simulink model "FSEA_Vehicle"  (R2026a)
settings: Solver=ode23tb  StopTime=5  FixedStep=.001  RelTol=1e-1
model workspace (MAT data in the model file):
  A_mu = 10
  B_reff = 8.386
  CONVERTER_DATA = [0 0.1 0.2 0.3 0.4 0.5 0.6 0.7 0.8 0.81 0.82 0.83 ... (63 elements, 21x3)]
  Cps = 2
  Cz = 7766.25
  DOWN_TABLE = [0 0 0 0 0 0 5 5 7.5 7.5 15 15 ... (30 elements, 6x5)]
  DOWN_TH_BP = [0 5 40 50 90 100]
  D_reff = 0.25826
  EMAP = [-40 215 245 264 264 267 267 267 267 267 -44 117 ... (110 elements, 10x11)]
  F0z = [6086.4 4324.8]
  F_reff = 0.07394
  F_zmax = 10000
  F_zmin = 100
  F_zo = 4000
  Kz = 48000
  MF : object (value not decoded)
  NCyl = 6
  NE_VEC = [800 1200 1600 2000 2400 2800 3200 3600 4000 4400 4800]
  Pstd = 101325
  Rair = 287
  SUS : object (value not decoded)
  TH_VEC = [0; 20; 30; 40; 50; 60; 70; 80; 90; 100]
  TWAITdn = 1.25
  TWAITup = 0.1
  Tin = [1 2 3 4 5 6 7 8 9 10 2 2 ... (20 elements, 10x2)]
  Tstd = 293.15
  UP_TABLE = [7.5 7.5 15 25 40 40 25 25 35 45 70 80 ... (30 elements, 6x5)]
  UP_TH_BP = [0 25 35 50 90 100]
  VEH : object (value not decoded)
  V_o = 16.7
  V_xlow = 1
  Vd = 0.00346
  WH : object (value not decoded)
  a = 1.515
  alpha_max = 1.5
  alpha_min = -1.5
  b = 1.504
  c_zo = 209651
  epsilon = 0.1
  f_air = [0 0 0 0 0 0 0 0 0 0 0 0 ... (256 elements, 16x16)]
  f_co = [0 0 0 0 0 0 0 0 0 0 0 0 ... (256 elements, 16x16)]
  f_co2 = [0 0 0 0 0 0 0 0 0 0 0 0 ... (256 elements, 16x16)]
  f_eff = [352.135682859 352.135682859 320.724378192 303.655312657 295.930136708 291.240087194 291.240271258 291.240312459 291.240275452 291.240198499 291.240100781 291.240018769 ... (256 elements, 16x16)]
  f_fuel = [0 0 0 0 0 0 0 0 0 0 0 0 ... (256 elements, 16x16)]
  f_hc = [0 0 0 0 0 0 0 0 0 0 0 0 ... (256 elements, 16x16)]
  f_nox = [0 0 0 0 0 0 0 0 0 0 0 0 ... (256 elements, 16x16)]
  f_pm = [0 0 0 0 0 0 0 0 0 0 0 0 ... (256 elements, 16x16)]
  f_susp_axl_bp = [1 2]
  f_susp_dz_bp = [-4 -0.14 -0.13 -0.12 -0.11 -0.1 -0.09 -0.08 -0.07 -0.06 -0.05 -0.04 ... (31 elements, 1x31)]
  f_susp_dzdot_bp = [-4 -0.14 -0.13 -0.12 -0.11 -0.1 -0.09 -0.08 -0.07 -0.06 -0.05 -0.04 ... (31 elements, 1x31)]
  f_susp_fmz = [-213379.591456 -28099.591456 -27619.591456 -27139.591456 -26659.591456 -26179.591456 -25699.591456 -25219.591456 -24739.591456 -24259.591456 -23779.591456 -23299.591456 ... (468968 elements, 31x31x61x2x4)]
  f_susp_geom = [-0.832564012244 0.043269987756 0.045538987756 0.047807987756 0.050076987756 0.052345987756 0.054614987756 0.056883987756 0.059152987756 0.061421987756 0.063690987756 0.065959987756 ... (11346 elements, 31x61x2x3)]
  f_susp_strgdelta_bp = [-0.523598775598 -0.506145483078 -0.488692190558 -0.471238898038 -0.453785605519 -0.436332312999 -0.418879020479 -0.401425727959 -0.383972435439 -0.366519142919 -0.349065850399 -0.331612557879 ... (61 elements, 1x61)]
  f_tbrake = [0 76.8593923996 105.140482948 131.533638111 157.926793274 176.658631717 176.65727296 176.656856686 176.656879077 176.657093756 176.657404516 176.65772406 ... (256 elements, 16x16)]
  f_tbrake_n_bpt = [0 649.519052838 912.419621844 1175.32019085 1438.22075986 1701.12132886 1964.02189787 2226.92246687 2489.82303588 2752.72360489 3015.62417389 3278.5247429 ... (16 elements, 1x16)]
  f_tbrake_t_bpt = [0 34.6410161514 61.0341713143 87.4273264773 113.82048164 140.213636803 166.606791966 192.999947129 219.393102292 245.786257455 272.179412618 298.572567781 ... (16 elements, 1x16)]
  f_texh = [766.752464599 766.752464599 786.17542386 801.679939032 884.591982581 910.574397722 910.571871054 910.570774534 910.570601632 910.570821151 910.571247242 910.571639815 ... (256 elements, 16x16)]
  f_twc_eff_co = [0.17 0.25 0.45 0.99 0.99 0.99 0.99]
  f_twc_eff_hc = [0.21 0.375 0.75 0.98 0.98 0.98 0.98]
  f_twc_eff_lam = [0.909090909 0.944055944 0.979020979 1 1.013986014 1.048951049 1.083916084]
  f_twc_eff_nox = [0.98 0.98 0.98 0.97 0.05 0.02 0]
  h = 0.134
  k_z = 50
  kappa_max = 1.5
  kappa_min = -1.5
  lam_Cx = 1
  lam_Cy = 1
  lam_Cz = 1
  lam_Ex = 1
  lam_Ey = 1
  lam_F_zo = 1
  lam_Hx = 1
  lam_Hy = 1
  lam_Kxkappa = 1
  lam_Kyalpha = 1
  lam_Kygamma = 1
  lam_Kzgamma = 1
  lam_Mr = 1
  lam_Mx = 1
  lam_My = 1
  lam_S = 1
  lam_VMx = 1
  lam_Vx = 1
  lam_Vy = 1
  lam_Vykappa = 1
  lam_muV = 0
  lam_mux = 1
  lam_muy = 1
  lam_t = 1
  lam_xalpha = 1
  lam_ykappa = 1
  numWheel = 4
  p_Cx1 = 1.579
  p_Cy1 = 1.3332
  p_Dx1 = 1.0422
  p_Dx2 = -0.08285
  p_Dx3 = 0
  p_Dy1 = 0.8784
  p_Dy2 = -0.06445
  p_Dy3 = 0
  p_Ex1 = 0.11185
  p_Ex2 = 0.3127
  p_Ex3 = 0
  p_Ex4 = 0.001603
  p_Ey1 = -0.8227
  p_Ey2 = -0.6062
  p_Ey3 = 0.09825
  p_Ey4 = -6.546
  p_Ey5 = 0
  p_Fz1 = 0.7098
  p_Hx1 = 0.00021585
  p_Hx2 = 0.0011538
  p_Hy1 = -0.0018043
  p_Hy2 = 0.003518
  p_Kx1 = 21.69
  p_Kx2 = 13.774
  p_Kx3 = -0.4119
  p_Ky1 = -15.314
  p_Ky2 = 1.7044
  p_Ky3 = 0.36986
  p_Ky4 = 1.9896
  p_Ky5 = 0
  p_Ky6 = -0.9004
  p_Ky7 = -0.2328
  p_Vx1 = 1.5973e-05
  p_Vx2 = 0.0001043
  p_Vy1 = -0.006642
  p_Vy2 = 0.03597
  p_Vy3 = -0.1621
  p_Vy4 = -0.4908
  p_pmx1 = 0
  p_px1 = -0.3489
  p_px2 = 0.382
  p_px3 = -0.09634
  p_px4 = 0.06447
  p_py1 = -0.6249
  p_py2 = -0.06535
  p_py3 = -0.1668
  p_py4 = 0.2834
  p_py5 = 0
  path : object (value not decoded)
  pio = 220000
  q_Fcx = 0
  q_Fz2 = 15.4
  q_Fzy = 0
  q_reo = 0.9974
  q_sx1 = -0.007764
  q_sx10 = 0.2824
  q_sx11 = 5.349
  q_sx12 = 0
  q_sx13 = 0
  q_sx14 = 0
  q_sx2 = 1.1915
  q_sx3 = 0.013948
  q_sx4 = 4.912
  q_sx5 = 1.02
  q_sx6 = 22.83
  q_sx7 = 0.7104
  q_sx8 = -0.023393
  q_sx9 = 0.6581
  q_sy1 = 0.00702
  q_sy2 = 0
  q_sy3 = 0.001515
  q_sy4 = 8.514e-05
  q_sy5 = 0
  q_sy6 = 0
  q_sy7 = 0.9008
  q_sy8 = -0.4089
  q_v1 = 0.0007742
  q_v2 = 0.04667
  r_Bx1 = 12.531
  r_Bx2 = 9.532
  r_Bx3 = 0
  r_By1 = 10.615
  r_By2 = 7.705
  r_By3 = 3.433e-06
  r_By4 = 0
  r_Cx1 = 1.019
  r_Cy1 = 1.0585
  r_Ex1 = -0.4487
  r_Ex2 = -0.4726
  r_Ey1 = 0.3132
  r_Ey2 = 7.63e-06
  r_Hx1 = 0.0002374
  r_Hy1 = 0.011646
  r_Hy2 = 7.63e-06
  r_Vy1 = 0.05654
  r_Vy2 = 7.63e-06
  r_Vy3 = 0
  r_Vy4 = 99.9
  r_Vy5 = 2
  r_Vy6 = 15.814
  r_o = 0.3135
  reqTmaxT = [nan 0.285774810084 0.647179872268 nan nan nan nan nan nan nan nan nan ... (168 elements, 21x8)]
  vehSpd = [0 2.77777777778 5.55555555556 8.33333333333 11.1111111111 13.8888888889 16.6666666667 19.4444444444 22.2222222222 25 27.7777777778 30.5555555556 ... (21 elements, 1x21)]
  vehWidth = 2
  w = 1
symbols that are objects in the model workspace (value not decoded): VEH
undefined symbols (not defined in the file or in its folder): InertFrm
libraries: sharedtransform x6, vehdynlibtirecommon x2, vehdynlibtire x2, autolibutils x2, autolibshared x2
(part 3 of 4)

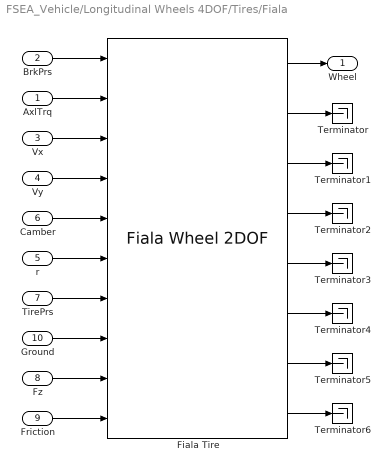
== system FSEA_Vehicle/Longitudinal Wheels 4DOF/Tires/Fiala ==
  AxlTrq : Inport
  BrkPrs : Inport  Port=2
  Vx : Inport  Port=3
  Vy : Inport  Port=4
  r : Inport  Port=5
  Camber : Inport  Port=6
  TirePrs : Inport  Port=7
  Fz : Inport  Port=8
  Friction : Inport  Port=9
  Ground : Inport  Port=10
  Fiala Tire : vehdynlibtire/Fiala Wheel 2DOF  tireType=Mid-size passenger car 235/45R18  BrakeType=Disc  rollingType=Pressure and velocity  vertType=None  Ckappa=217325.388  Calpha=104298.5693  Cgamma=-3413.1559  muMin=0.17601  muMax=1.3803  Lrelx=.01  Lrely=.01  NOMPRES=220000  LONGVL=16  aMy=8e-4  bMy=.001  cMy=1.6e-4  alphaMy=-0.003  betaMy=0.97  QSY1=0.007  QSY2=0  QSY3=0.0015  QSY4=8.5e-05  QSY5=0  QSY6=0  QSY7=0.9  QSY8=-0.4  FNOMIN=4000  lam_My=1  VxMy=-20:1:20  FzMy=0:200:1e4  MyMap=|  Fpl=10  Cr=1e-3  Kt=.008  Tmeas=298.15  Tamb=298.15  extTamb=off  WIDTH=0.235  bMz=0  mu_static=.3  mu_kinetic=.2  disk_abore=.05  Rm=.177  num_pads=2  drum_abore=0.0508  drum_a=0.123  drum_c=0.212  drum_r=0.15  drum_theta1=0  drum_theta2=126  brake_p_bpt=[1 11.4736842105263 21.9473684210526 32.4210526315789 42.8947368421053 53.3684210526316 63.8421052631579 74.3157894736842 84.7894736842105 95.2631578947368 105.736842105263 116.210526315789 126.684210526316 137.157894736842 147.631578947368 158.105263157895 168.578947368421 179.052631578947 189.526315789474 200]  brake_n_bpt=[0 52.6315789473684 105.263157894737 157.894736842105 210.526315789474 263.157894736842 315.789473684211 368.421052631579 421.052631578947 473.684210526316 526.315789473684 578.947368421053 631.578947368421 684.210526315789 736.842105263158 789.473684210526 842.105263157895 894.736842105263 947.368421052632 1000]  f_brake_t=[43.4900602404453 42.5056030554862 41.5350898940194 40.5780454442085 39.6340111501808 38.7025443887544 37.7832176914519 36.8756180088306 35.9793460143796 35.0940154454303 34.2192524787115 33.3546951383474 32.4999927342521 31.6548053290159 30.8188032315107 29.991666515561 29.1730845621415 28.362755623661 27.5603864089927 26.765691687993;498.991217495636 487.695866636631 476.560505099801 465.579679307235 454.748127933653 444.060772460445 433.51270824929 423.099196101319 412.81565427025 402.657650900201 392.620896861006 382.701238955775 372.894653477208 363.197240090814 353.605216024701 344.114910546964 334.722759712992 325.425301366216 316.219170376863 307.10109410434;954.492374750826 932.886130217776 911.585920305583 890.581313170261 869.862244717126 849.419000532136 829.242198807128 809.322774193808 789.651962526121 770.221286354971 751.0225412433 732.047782773203 713.289314220164 694.739674852612 676.391628817892 658.238154578366 640.272434863842 622.48784710877 604.877954344734 587.436496520688;1409.99353200602 1378.07639379892 1346.61133551136 1315.58294703329 1284.9763615006 1254.77722860383 1224.97168936497 1195.5463522863 1166.48827078199 1137.78492180974 1109.42418562559 1081.39432659063 1053.68397496312 1026.28210961441 999.178041611083 972.361398609768 945.822110014692 919.550392851325 893.536738312604 867.771898937035;1865.49468926121 1823.26665738007 1781.63675071715 1740.58458089631 1700.09047828407 1660.13545667552 1620.7011799228 1581.76993037878 1543.32457903786 1505.34855726451 1467.82583000789 1430.74087040806 1394.07863570608 1357.82454437621 1321.96445440427 1286.48464264117 1251.37178516554 1216.61293859388 1182.19552228048 1148.10730135338;2320.9958465164 2268.45692096121 2216.66216592293 2165.58621475934 2115.20459506754 2065.49368474721 2016.43067048064 1967.99350847127 1920.16088729373 1872.91219271928 1826.22747439018 1780.08741422549 1734.47329644903 1689.36697913801 1644.75086719747 1600.60788667257 1556.92146031639 1513.67548433643 1470.85430624835 1428.44270376973;2776.49700377159 2713.64718454235 2651.68758112871 2590.58784862237 2530.31871185102 2470.8519128189 2412.16016103848 2354.21708656376 2296.9971955496 2240.47582817405 2184.62911877248 2129.43395804292 2074.86795719199 2020.9094138998 1967.53727999066 1914.73113070398 1862.47113546724 1810.73803007899 1759.51309021622 1708.77810618608;3231.99816102678 3158.8374481235 3086.71299633449 3015.58948248539 2945.43282863449 2876.21014089059 2807.88965159632 2740.44066465625 2673.83350380547 2608.03946362882 2543.03076315477 2478.78050186034 2415.26261793494 2352.4518486616 2290.32369278385 2228.85437473538 2168.02081061809 2107.80057582154 2048.17187418409 1989.11350860242;3687.49931828197 3604.02771170464 3521.73841154027 3440.59111634842 3360.54694541796 3281.56836896228 3203.61914215416 3126.66424274874 3050.66981206134 2975.60309908359 2901.43240753707 2828.12704567777 2755.6572786779 2683.9942834234 2613.11010557704 2542.97761876678 2473.57048576894 2404.8631215641 2336.83065815196 2269.44891101877;4143.00047553716 4049.21797528579 3956.76382674606 3865.59275021144 3775.66106220143 3686.92659703397 3599.34863271199 3512.88782084123 3427.50612031721 3343.16673453836 3259.83405191936 3177.4735894952 3096.05193942085 3015.5367181852 2935.89651837023 2857.10086279818 2779.12016091979 2701.92566730665 2625.48944211983 2549.78431343512;4598.50163279235 4494.40823886693 4391.78924195184 4290.59438407447 4190.77517898491 4092.28482510566 3995.07812326983 3899.11139893372 3804.34242857308 3710.73036999313 3618.23569630166 3526.82013331263 3436.44660016381 3347.079152947 3258.68293116342 3171.22410682959 3084.66983607064 2998.98821304921 2914.1482260877 2830.11971585147;5054.00279004754 4939.59850244808 4826.81465715762 4715.59601793749 4605.88929576838 4497.64305317735 4390.80761382767 4285.3349770262 4181.17873682896 4078.2940054479 3976.63734068395 3876.16667713006 3776.84126090677 3678.62158770879 3581.46934395661 3485.34735086099 ...(+2764 chars)]  MASS=9.46491996974568  zo=0  zdoto=0  GRAVITY=-9.81  VERTICAL_STIFFNESS=207885  VERTICAL_DAMPING=500  zFz=[0 .01 .1]  pFz=[10000 1000000]  Fzz=[0 1e3 1e4; 0 1e4 1e5]  zdotFz=[-20 0 20]  Fzzdot=[500 0 -500;250 0 -250]  UNLOADED_RADIUS=0.33454  omegao=0  IYY=0.740633832792491  br=1e-3  FZMAX=8600  FZMIN=100  PRESMAX=1000000  PRESMIN=10000  KPUMAX=0.5  KPUMIN=-0.5  ALPMAX=0.7854  ALPMIN=-0.7854  CAMMAX=0.17453  CAMMIN=-0.17453  TMIN=0  TMAX=400  aMode=2  MyRelFreqLwrLim=100*pi
      | [0,1114.7,4367.1,9707.2,17109,26554,38030,51524,67028,84533,1.0403e+05,1.2552e+05,1.4899e+05,1.7444e+05,2.0185e+05,2.3124e+05,2.6259e+05,2.959e+05,3.3117e+05,3.6839e+05,4.0756e+05,4.4868e+05,4.9174e+05,5.3675e+05,5.8369e+05,6.3257e+05,6.8338e+05,7.3613e+05,7.908e+05,8.474e+05,9.0593e+05,9.6638e+05,1.0288e+06,1.093e+06,1.1593e+06,1.2274e+06,1.2974e+06,1.3694e+06,1.4432e+06,1.519e+06,1.5967e+06,1.6763e+06,1.7578e+06,1.8412e+06,1.9265e+06,2.0137e+06,2.1028e+06,2.1938e+06,2.2867e+06,2.3815e+06,2.4782e+06
      | 0,1024.5,4013.8,8921.9,15725,24406,34953,47356,61605,77694,95616,1.1537e+05,1.3694e+05,1.6032e+05,1.8553e+05,2.1254e+05,2.4135e+05,2.7197e+05,3.0438e+05,3.3859e+05,3.7459e+05,4.1238e+05,4.5196e+05,4.9333e+05,5.3647e+05,5.814e+05,6.281e+05,6.7658e+05,7.2683e+05,7.7885e+05,8.3264e+05,8.8821e+05,9.4553e+05,1.0046e+06,1.0655e+06,1.1281e+06,1.1925e+06,1.2586e+06,1.3265e+06,1.3961e+06,1.4675e+06,1.5407e+06,1.6156e+06,1.6922e+06,1.7706e+06,1.8508e+06,1.9327e+06,2.0163e+06,2.1017e+06,2.1889e+06,2.2777e+06
      | 0,938.57,3677,8173.3,14405,22358,32020,43382,56436,71175,87593,1.0568e+05,1.2545e+05,1.4687e+05,1.6996e+05,1.947e+05,2.211e+05,2.4915e+05,2.7884e+05,3.1018e+05,3.4316e+05,3.7778e+05,4.1404e+05,4.5193e+05,4.9146e+05,5.3261e+05,5.754e+05,6.1981e+05,6.6584e+05,7.135e+05,7.6278e+05,8.1368e+05,8.6619e+05,9.2032e+05,9.7607e+05,1.0334e+06,1.0924e+06,1.153e+06,1.2152e+06,1.279e+06,1.3444e+06,1.4114e+06,1.48e+06,1.5502e+06,1.6221e+06,1.6955e+06,1.7705e+06,1.8471e+06,1.9254e+06,2.0052e+06,2.0866e+06
      | 0,856.81,3356.7,7461.3,13151,20411,29231,39603,51520,64974,79962,96478,1.1452e+05,1.3408e+05,1.5515e+05,1.7774e+05,2.0184e+05,2.2744e+05,2.5455e+05,2.8316e+05,3.1327e+05,3.4487e+05,3.7797e+05,4.1256e+05,4.4864e+05,4.8621e+05,5.2527e+05,5.6581e+05,6.0784e+05,6.5134e+05,6.9633e+05,7.4279e+05,7.9073e+05,8.4015e+05,8.9104e+05,9.4341e+05,9.9724e+05,1.0525e+06,1.1093e+06,1.1676e+06,1.2273e+06,1.2885e+06,1.3511e+06,1.4152e+06,1.4808e+06,1.5478e+06,1.6163e+06,1.6862e+06,1.7576e+06,1.8305e+06,1.9048e+06
      | 0,779.25,3052.9,6785.9,11960,18563,26585,36018,46856,59093,72724,87745,1.0415e+05,1.2194e+05,1.4111e+05,1.6165e+05,1.8357e+05,2.0685e+05,2.3151e+05,2.5753e+05,2.8491e+05,3.1365e+05,3.4376e+05,3.7522e+05,4.0803e+05,4.422e+05,4.7772e+05,5.1459e+05,5.5282e+05,5.9238e+05,6.333e+05,6.7556e+05,7.1916e+05,7.641e+05,8.1039e+05,8.5801e+05,9.0697e+05,9.5727e+05,1.0089e+06,1.0619e+06,1.1162e+06,1.1718e+06,1.2288e+06,1.2871e+06,1.3467e+06,1.4077e+06,1.47e+06,1.5336e+06,1.5985e+06,1.6648e+06,1.7324e+06
      | 0,705.9,2765.5,6147.1,10834,16816,24083,32628,42446,53531,65879,79486,94348,1.1046e+05,1.2783e+05,1.4643e+05,1.6629e+05,1.8738e+05,2.0972e+05,2.3329e+05,2.5809e+05,2.8413e+05,3.114e+05,3.399e+05,3.6962e+05,4.0058e+05,4.3276e+05,4.6616e+05,5.0078e+05,5.3662e+05,5.7369e+05,6.1197e+05,6.5146e+05,6.9218e+05,7.3411e+05,7.7725e+05,8.216e+05,8.6717e+05,9.1394e+05,9.6193e+05,1.0111e+06,1.0615e+06,1.1131e+06,1.1659e+06,1.22e+06,1.2752e+06,1.3316e+06,1.3892e+06,1.4481e+06,1.5081e+06,1.5693e+06
      | 0,636.76,2494.6,5545,9773.1,15169,21724,29432,38288,48287,59426,71700,85106,99642,1.153e+05,1.3209e+05,1.5e+05,1.6903e+05,1.8917e+05,2.1044e+05,2.3281e+05,2.563e+05,2.809e+05,3.066e+05,3.3342e+05,3.6134e+05,3.9037e+05,4.205e+05,4.5173e+05,4.8406e+05,5.1749e+05,5.5202e+05,5.8765e+05,6.2438e+05,6.622e+05,7.0111e+05,7.4112e+05,7.8223e+05,8.2442e+05,8.677e+05,9.1208e+05,9.5754e+05,1.0041e+06,1.0517e+06,1.1005e+06,1.1503e+06,1.2012e+06,1.2532e+06,1.3062e+06,1.3604e+06,1.4156e+06
      | 0,571.82,2240.2,4979.5,8776.4,13622,19508,26430,34383,43363,53365,64388,76427,89480,1.0355e+05,1.1862e+05,1.347e+05,1.5179e+05,1.6988e+05,1.8897e+05,2.0907e+05,2.3016e+05,2.5225e+05,2.7534e+05,2.9942e+05,3.2449e+05,3.5056e+05,3.7761e+05,4.0566e+05,4.3469e+05,4.6472e+05,4.9573e+05,5.2772e+05,5.607e+05,5.9467e+05,6.2961e+05,6.6554e+05,7.0245e+05,7.4034e+05,7.7921e+05,8.1906e+05,8.5989e+05,9.017e+05,9.4448e+05,9.8824e+05,1.033e+06,1.0787e+06,1.1254e+06,1.173e+06,1.2216e+06,1.2712e+06
      | 0,511.09,2002.3,4450.7,7844.3,12175,17436,23623,30732,38757,47698,57549,68310,79977,92548,1.0602e+05,1.204e+05,1.3567e+05,1.5184e+05,1.689e+05,1.8686e+05,2.0572e+05,2.2546e+05,2.4609e+05,2.6762e+05,2.9003e+05,3.1332e+05,3.3751e+05,3.6258e+05,3.8853e+05,4.1536e+05,4.4308e+05,4.7167e+05,5.0115e+05,5.3151e+05,5.6274e+05,5.9486e+05,6.2785e+05,6.6171e+05,6.9646e+05,7.3207e+05,7.6857e+05,8.0593e+05,8.4417e+05,8.8328e+05,9.2326e+05,9.6412e+05,1.0058e+06,1.0484e+06,1.0919e+06,1.1362e+06
      | 0,454.56,1780.8,3958.4,6976.8,10828,15508,21011,27333,34471,42422,51185,60755,71132,82313,94296,1.0708e+05,1.2066e+05,1.3505e+05,1.5022e+05,1.662e+05,1.8296e+05,2.0052e+05,2.1888e+05,2.3802e+05,2.5795e+05,2.7867e+05,3.0018e+05,3.2248e+05,3.4556e+05,3.6942e+05,3.9407e+05,4.1951e+05,4.4573e+05,4.7273e+05,5.0051e+05,5.2907e+05,5.5841e+05,5.8853e+05,6.1943e+05,6.5111e+05,6.8356e+05,7.168e+05,7.5081e+05,7.8559e+05,8.2115e+05,8.5749e+05,8.946e+05,9.3248e+05,9.7114e+05,1.0106e+06
      | 0,402.25,1575.9,3502.8,6173.8,9582.1,13723,18592,24187,30503,37540,45293,53762,62945,72839,83443,94756,1.0678e+05,1.195e+05,1.3293e+05,1.4707e+05,1.6191e+05,1.7745e+05,1.9368e+05,2.1062e+05,2.2826e+05,2.466e+05,2.6563e+05,2.8536e+05,3.0578e+05,3.269e+05,3.4872e+05,3.7123e+05,3.9442e+05,4.1832e+05,4.429e+05,4.6817e+05,4.9414e+05,5.2079e+05,5.4814e+05,5.7617e+05,6.0489e+05,6.343e+05,6.6439e+05,6.9517e+05,7.2664e+05,7.588e+05,7.9163e+05,8.2516e+05,8.5937e+05,8.9426e+05
      | 0,354.13,1387.4,3083.9,5435.3,8436,12082,16369,21294,26855,33050,39876,47332,55416,64127,73463,83423,94005,1.0521e+05,1.1703e+05,1.2948e+05,1.4254e+05,1.5622e+05,1.7052e+05,1.8543e+05,2.0096e+05,2.171e+05,2.3386e+05,2.5123e+05,2.6921e+05,2.878e+05,3.0701e+05,3.2682e+05,3.4725e+05,3.6828e+05,3.8993e+05,4.1218e+05,4.3504e+05,4.585e+05,4.8258e+05,5.0725e+05,5.3254e+05,5.5843e+05,5.8493e+05,6.1203e+05,6.3973e+05,6.6804e+05,6.9695e+05,7.2646e+05,7.5658e+05,7.873e+05
      | 0,310.23,1215.4,2701.5,4761.5,7390.2,10584,14339,18654,23526,28952,34932,41464,48546,56176,64355,73080,82351,92166,1.0252e+05,1.1343e+05,1.2487e+05,1.3685e+05,1.4938e+05,1.6244e+05,1.7605e+05,1.9019e+05,2.0487e+05,2.2008e+05,2.3583e+05,2.5212e+05,2.6895e+05,2.863e+05,3.042e+05,3.2262e+05,3.4158e+05,3.6108e+05,3.811e+05,4.0166e+05,4.2275e+05,4.4437e+05,4.6652e+05,4.892e+05,5.1241e+05,5.3615e+05,5.6042e+05,5.8521e+05,6.1054e+05,6.364e+05,6.6278e+05,6.8969e+05
      | 0,270.53,1059.9,2355.8,4152.2,6444.5,9229.4,12504,16267,20515,25247,30462,36158,42334,48988,56120,63728,71813,80372,89405,98911,1.0889e+05,1.1934e+05,1.3026e+05,1.4166e+05,1.5352e+05,1.6585e+05,1.7865e+05,1.9192e+05,2.0566e+05,2.1986e+05,2.3453e+05,2.4967e+05,2.6527e+05,2.8134e+05,2.9787e+05,3.1487e+05,3.3233e+05,3.5026e+05,3.6865e+05,3.875e+05,4.0682e+05,4.266e+05,4.4684e+05,4.6754e+05,4.887e+05,5.1033e+05,5.3241e+05,5.5496e+05,5.7797e+05,6.0143e+05
      | 0,235.04,920.8,2046.8,3607.4,5599,8018.6,10864,14133,17824,21935,26466,31414,36780,42561,48757,55367,62391,69827,77675,85934,94604,1.0368e+05,1.1317e+05,1.2307e+05,1.3338e+05,1.4409e+05,1.5521e+05,1.6674e+05,1.7867e+05,1.9101e+05,2.0376e+05,2.1691e+05,2.3047e+05,2.4443e+05,2.5879e+05,2.7356e+05,2.8873e+05,3.0431e+05,3.2028e+05,3.3666e+05,3.5345e+05,3.7063e+05,3.8821e+05,4.062e+05,4.2459e+05,4.4337e+05,4.6256e+05,4.8215e+05,5.0214e+05,5.2253e+05
      | 0,203.75,798.24,1774.3,3127.2,4853.7,6951.2,9417.7,12252,15451,19015,22943,27233,31884,36896,42267,47997,54086,60533,67336,74496,82011,89882,98108,1.0669e+05,1.1562e+05,1.2491e+05,1.3455e+05,1.4455e+05,1.5489e+05,1.6559e+05,1.7664e+05,1.8804e+05,1.9979e+05,2.1189e+05,2.2434e+05,2.3715e+05,2.503e+05,2.638e+05,2.7765e+05,2.9185e+05,3.064e+05,3.2129e+05,3.3654e+05,3.5213e+05,3.6807e+05,3.8436e+05,4.0099e+05,4.1797e+05,4.353e+05,4.5297e+05
      | 0,176.67,692.15,1538.5,2711.6,4208.6,6027.4,8166.1,10623,13398,16488,19894,23613,27646,31992,36650,41618,46898,52488,58387,64595,71112,77937,85069,92509,1.0026e+05,1.0831e+05,1.1667e+05,1.2533e+05,1.3431e+05,1.4358e+05,1.5316e+05,1.6305e+05,1.7324e+05,1.8373e+05,1.9453e+05,2.0563e+05,2.1703e+05,2.2874e+05,2.4075e+05,2.5306e+05,2.6568e+05,2.7859e+05,2.9181e+05,3.0533e+05,3.1915e+05,3.3327e+05,3.477e+05,3.6242e+05,3.7745e+05,3.9277e+05
      | 0,153.8,602.54,1339.3,2360.6,3663.8,5247,7108.9,9247.9,11663,14353,17318,20556,24067,27850,31905,36230,40826,45692,50828,56232,61905,67847,74056,80533,87277,94287,1.0156e+05,1.0911e+05,1.1692e+05,1.2499e+05,1.3333e+05,1.4194e+05,1.5081e+05,1.5994e+05,1.6934e+05,1.7901e+05,1.8894e+05,1.9913e+05,2.0958e+05,2.203e+05,2.3128e+05,2.4253e+05,2.5403e+05,2.658e+05,2.7783e+05,2.9013e+05,3.0268e+05,3.155e+05,3.2858e+05,3.4192e+05
      | 0,135.13,529.41,1176.8,2074.1,3219.1,4610.2,6246.1,8125.5,10248,12611,15216,18061,21146,24470,28033,31833,35871,40147,44659,49407,54392,59612,65068,70759,76684,82844,89238,95866,1.0273e+05,1.0982e+05,1.1715e+05,1.2471e+05,1.3251e+05,1.4053e+05,1.4879e+05,1.5728e+05,1.66e+05,1.7496e+05,1.8415e+05,1.9356e+05,2.0321e+05,2.1309e+05,2.232e+05,2.3354e+05,2.4411e+05,2.5492e+05,2.6595e+05,2.7721e+05,2.887e+05,3.0042e+05
      | 0,120.67,472.76,1050.9,1852.1,2874.6,4116.9,5577.7,7256.1,9151,11262,13588,16129,18883,21852,25033,28427,32033,35851,39880,44121,48572,53234,58105,63187,68479,73979,79689,85608,91735,98071,1.0462e+05,1.1137e+05,1.1833e+05,1.255e+05,1.3287e+05,1.4045e+05,1.4824e+05,1.5624e+05,1.6444e+05,1.7285e+05,1.8147e+05,1.9029e+05,1.9932e+05,2.0855e+05,2.1799e+05,2.2764e+05,2.3749e+05,2.4755e+05,2.5781e+05,2.6828e+05
      | 0,110.42,432.59,961.56,1694.8,2630.4,3767.1,5103.8,6639.5,8373.5,10305,12433,14758,17279,19995,22906,26012,29311,32805,36492,40372,44445,48710,53168,57818,62660,67694,72918,78334,83941,89738,95727,1.019e+05,1.0827e+05,1.1483e+05,1.2158e+05,1.2852e+05,1.3565e+05,1.4296e+05,1.5047e+05,1.5816e+05,1.6605e+05,1.7412e+05,1.8238e+05,1.9083e+05,1.9947e+05,2.083e+05,2.1731e+05,2.2651e+05,2.359e+05,2.4548e+05
      | 0,120.67,472.76,1050.9,1852.1,2874.6,4116.9,5577.7,7256.1,9151,11262,13588,16129,18883,21852,25033,28427,32033,35851,39880,44121,48572,53234,58105,63187,68479,73979,79689,85608,91735,98071,1.0462e+05,1.1137e+05,1.1833e+05,1.255e+05,1.3287e+05,1.4045e+05,1.4824e+05,1.5624e+05,1.6444e+05,1.7285e+05,1.8147e+05,1.9029e+05,1.9932e+05,2.0855e+05,2.1799e+05,2.2764e+05,2.3749e+05,2.4755e+05,2.5781e+05,2.6828e+05
      | 0,135.13,529.41,1176.8,2074.1,3219.1,4610.2,6246.1,8125.5,10248,12611,15216,18061,21146,24470,28033,31833,35871,40147,44659,49407,54392,59612,65068,70759,76684,82844,89238,95866,1.0273e+05,1.0982e+05,1.1715e+05,1.2471e+05,1.3251e+05,1.4053e+05,1.4879e+05,1.5728e+05,1.66e+05,1.7496e+05,1.8415e+05,1.9356e+05,2.0321e+05,2.1309e+05,2.232e+05,2.3354e+05,2.4411e+05,2.5492e+05,2.6595e+05,2.7721e+05,2.887e+05,3.0042e+05
      | 0,153.8,602.54,1339.3,2360.6,3663.8,5247,7108.9,9247.9,11663,14353,17318,20556,24067,27850,31905,36230,40826,45692,50828,56232,61905,67847,74056,80533,87277,94287,1.0156e+05,1.0911e+05,1.1692e+05,1.2499e+05,1.3333e+05,1.4194e+05,1.5081e+05,1.5994e+05,1.6934e+05,1.7901e+05,1.8894e+05,1.9913e+05,2.0958e+05,2.203e+05,2.3128e+05,2.4253e+05,2.5403e+05,2.658e+05,2.7783e+05,2.9013e+05,3.0268e+05,3.155e+05,3.2858e+05,3.4192e+05
      | 0,176.67,692.15,1538.5,2711.6,4208.6,6027.4,8166.1,10623,13398,16488,19894,23613,27646,31992,36650,41618,46898,52488,58387,64595,71112,77937,85069,92509,1.0026e+05,1.0831e+05,1.1667e+05,1.2533e+05,1.3431e+05,1.4358e+05,1.5316e+05,1.6305e+05,1.7324e+05,1.8373e+05,1.9453e+05,2.0563e+05,2.1703e+05,2.2874e+05,2.4075e+05,2.5306e+05,2.6568e+05,2.7859e+05,2.9181e+05,3.0533e+05,3.1915e+05,3.3327e+05,3.477e+05,3.6242e+05,3.7745e+05,3.9277e+05
      | 0,203.75,798.24,1774.3,3127.2,4853.7,6951.2,9417.7,12252,15451,19015,22943,27233,31884,36896,42267,47997,54086,60533,67336,74496,82011,89882,98108,1.0669e+05,1.1562e+05,1.2491e+05,1.3455e+05,1.4455e+05,1.5489e+05,1.6559e+05,1.7664e+05,1.8804e+05,1.9979e+05,2.1189e+05,2.2434e+05,2.3715e+05,2.503e+05,2.638e+05,2.7765e+05,2.9185e+05,3.064e+05,3.2129e+05,3.3654e+05,3.5213e+05,3.6807e+05,3.8436e+05,4.0099e+05,4.1797e+05,4.353e+05,4.5297e+05
      | 0,235.04,920.8,2046.8,3607.4,5599,8018.6,10864,14133,17824,21935,26466,31414,36780,42561,48757,55367,62391,69827,77675,85934,94604,1.0368e+05,1.1317e+05,1.2307e+05,1.3338e+05,1.4409e+05,1.5521e+05,1.6674e+05,1.7867e+05,1.9101e+05,2.0376e+05,2.1691e+05,2.3047e+05,2.4443e+05,2.5879e+05,2.7356e+05,2.8873e+05,3.0431e+05,3.2028e+05,3.3666e+05,3.5345e+05,3.7063e+05,3.8821e+05,4.062e+05,4.2459e+05,4.4337e+05,4.6256e+05,4.8215e+05,5.0214e+05,5.2253e+05
      | 0,270.53,1059.9,2355.8,4152.2,6444.5,9229.4,12504,16267,20515,25247,30462,36158,42334,48988,56120,63728,71813,80372,89405,98911,1.0889e+05,1.1934e+05,1.3026e+05,1.4166e+05,1.5352e+05,1.6585e+05,1.7865e+05,1.9192e+05,2.0566e+05,2.1986e+05,2.3453e+05,2.4967e+05,2.6527e+05,2.8134e+05,2.9787e+05,3.1487e+05,3.3233e+05,3.5026e+05,3.6865e+05,3.875e+05,4.0682e+05,4.266e+05,4.4684e+05,4.6754e+05,4.887e+05,5.1033e+05,5.3241e+05,5.5496e+05,5.7797e+05,6.0143e+05
      | 0,310.23,1215.4,2701.5,4761.5,7390.2,10584,14339,18654,23526,28952,34932,41464,48546,56176,64355,73080,82351,92166,1.0252e+05,1.1343e+05,1.2487e+05,1.3685e+05,1.4938e+05,1.6244e+05,1.7605e+05,1.9019e+05,2.0487e+05,2.2008e+05,2.3583e+05,2.5212e+05,2.6895e+05,2.863e+05,3.042e+05,3.2262e+05,3.4158e+05,3.6108e+05,3.811e+05,4.0166e+05,4.2275e+05,4.4437e+05,4.6652e+05,4.892e+05,5.1241e+05,5.3615e+05,5.6042e+05,5.8521e+05,6.1054e+05,6.364e+05,6.6278e+05,6.8969e+05
      | 0,354.13,1387.4,3083.9,5435.3,8436,12082,16369,21294,26855,33050,39876,47332,55416,64127,73463,83423,94005,1.0521e+05,1.1703e+05,1.2948e+05,1.4254e+05,1.5622e+05,1.7052e+05,1.8543e+05,2.0096e+05,2.171e+05,2.3386e+05,2.5123e+05,2.6921e+05,2.878e+05,3.0701e+05,3.2682e+05,3.4725e+05,3.6828e+05,3.8993e+05,4.1218e+05,4.3504e+05,4.585e+05,4.8258e+05,5.0725e+05,5.3254e+05,5.5843e+05,5.8493e+05,6.1203e+05,6.3973e+05,6.6804e+05,6.9695e+05,7.2646e+05,7.5658e+05,7.873e+05
      | 0,402.25,1575.9,3502.8,6173.8,9582.1,13723,18592,24187,30503,37540,45293,53762,62945,72839,83443,94756,1.0678e+05,1.195e+05,1.3293e+05,1.4707e+05,1.6191e+05,1.7745e+05,1.9368e+05,2.1062e+05,2.2826e+05,2.466e+05,2.6563e+05,2.8536e+05,3.0578e+05,3.269e+05,3.4872e+05,3.7123e+05,3.9442e+05,4.1832e+05,4.429e+05,4.6817e+05,4.9414e+05,5.2079e+05,5.4814e+05,5.7617e+05,6.0489e+05,6.343e+05,6.6439e+05,6.9517e+05,7.2664e+05,7.588e+05,7.9163e+05,8.2516e+05,8.5937e+05,8.9426e+05
      | 0,454.56,1780.8,3958.4,6976.8,10828,15508,21011,27333,34471,42422,51185,60755,71132,82313,94296,1.0708e+05,1.2066e+05,1.3505e+05,1.5022e+05,1.662e+05,1.8296e+05,2.0052e+05,2.1888e+05,2.3802e+05,2.5795e+05,2.7867e+05,3.0018e+05,3.2248e+05,3.4556e+05,3.6942e+05,3.9407e+05,4.1951e+05,4.4573e+05,4.7273e+05,5.0051e+05,5.2907e+05,5.5841e+05,5.8853e+05,6.1943e+05,6.5111e+05,6.8356e+05,7.168e+05,7.5081e+05,7.8559e+05,8.2115e+05,8.5749e+05,8.946e+05,9.3248e+05,9.7114e+05,1.0106e+06
      | 0,511.09,2002.3,4450.7,7844.3,12175,17436,23623,30732,38757,47698,57549,68310,79977,92548,1.0602e+05,1.204e+05,1.3567e+05,1.5184e+05,1.689e+05,1.8686e+05,2.0572e+05,2.2546e+05,2.4609e+05,2.6762e+05,2.9003e+05,3.1332e+05,3.3751e+05,3.6258e+05,3.8853e+05,4.1536e+05,4.4308e+05,4.7167e+05,5.0115e+05,5.3151e+05,5.6274e+05,5.9486e+05,6.2785e+05,6.6171e+05,6.9646e+05,7.3207e+05,7.6857e+05,8.0593e+05,8.4417e+05,8.8328e+05,9.2326e+05,9.6412e+05,1.0058e+06,1.0484e+06,1.0919e+06,1.1362e+06
      | 0,571.82,2240.2,4979.5,8776.4,13622,19508,26430,34383,43363,53365,64388,76427,89480,1.0355e+05,1.1862e+05,1.347e+05,1.5179e+05,1.6988e+05,1.8897e+05,2.0907e+05,2.3016e+05,2.5225e+05,2.7534e+05,2.9942e+05,3.2449e+05,3.5056e+05,3.7761e+05,4.0566e+05,4.3469e+05,4.6472e+05,4.9573e+05,5.2772e+05,5.607e+05,5.9467e+05,6.2961e+05,6.6554e+05,7.0245e+05,7.4034e+05,7.7921e+05,8.1906e+05,8.5989e+05,9.017e+05,9.4448e+05,9.8824e+05,1.033e+06,1.0787e+06,1.1254e+06,1.173e+06,1.2216e+06,1.2712e+06
      | 0,636.76,2494.6,5545,9773.1,15169,21724,29432,38288,48287,59426,71700,85106,99642,1.153e+05,1.3209e+05,1.5e+05,1.6903e+05,1.8917e+05,2.1044e+05,2.3281e+05,2.563e+05,2.809e+05,3.066e+05,3.3342e+05,3.6134e+05,3.9037e+05,4.205e+05,4.5173e+05,4.8406e+05,5.1749e+05,5.5202e+05,5.8765e+05,6.2438e+05,6.622e+05,7.0111e+05,7.4112e+05,7.8223e+05,8.2442e+05,8.677e+05,9.1208e+05,9.5754e+05,1.0041e+06,1.0517e+06,1.1005e+06,1.1503e+06,1.2012e+06,1.2532e+06,1.3062e+06,1.3604e+06,1.4156e+06
      | 0,705.9,2765.5,6147.1,10834,16816,24083,32628,42446,53531,65879,79486,94348,1.1046e+05,1.2783e+05,1.4643e+05,1.6629e+05,1.8738e+05,2.0972e+05,2.3329e+05,2.5809e+05,2.8413e+05,3.114e+05,3.399e+05,3.6962e+05,4.0058e+05,4.3276e+05,4.6616e+05,5.0078e+05,5.3662e+05,5.7369e+05,6.1197e+05,6.5146e+05,6.9218e+05,7.3411e+05,7.7725e+05,8.216e+05,8.6717e+05,9.1394e+05,9.6193e+05,1.0111e+06,1.0615e+06,1.1131e+06,1.1659e+06,1.22e+06,1.2752e+06,1.3316e+06,1.3892e+06,1.4481e+06,1.5081e+06,1.5693e+06
      | 0,779.25,3052.9,6785.9,11960,18563,26585,36018,46856,59093,72724,87745,1.0415e+05,1.2194e+05,1.4111e+05,1.6165e+05,1.8357e+05,2.0685e+05,2.3151e+05,2.5753e+05,2.8491e+05,3.1365e+05,3.4376e+05,3.7522e+05,4.0803e+05,4.422e+05,4.7772e+05,5.1459e+05,5.5282e+05,5.9238e+05,6.333e+05,6.7556e+05,7.1916e+05,7.641e+05,8.1039e+05,8.5801e+05,9.0697e+05,9.5727e+05,1.0089e+06,1.0619e+06,1.1162e+06,1.1718e+06,1.2288e+06,1.2871e+06,1.3467e+06,1.4077e+06,1.47e+06,1.5336e+06,1.5985e+06,1.6648e+06,1.7324e+06
      | 0,856.81,3356.7,7461.3,13151,20411,29231,39603,51520,64974,79962,96478,1.1452e+05,1.3408e+05,1.5515e+05,1.7774e+05,2.0184e+05,2.2744e+05,2.5455e+05,2.8316e+05,3.1327e+05,3.4487e+05,3.7797e+05,4.1256e+05,4.4864e+05,4.8621e+05,5.2527e+05,5.6581e+05,6.0784e+05,6.5134e+05,6.9633e+05,7.4279e+05,7.9073e+05,8.4015e+05,8.9104e+05,9.4341e+05,9.9724e+05,1.0525e+06,1.1093e+06,1.1676e+06,1.2273e+06,1.2885e+06,1.3511e+06,1.4152e+06,1.4808e+06,1.5478e+06,1.6163e+06,1.6862e+06,1.7576e+06,1.8305e+06,1.9048e+06
      | 0,938.57,3677,8173.3,14405,22358,32020,43382,56436,71175,87593,1.0568e+05,1.2545e+05,1.4687e+05,1.6996e+05,1.947e+05,2.211e+05,2.4915e+05,2.7884e+05,3.1018e+05,3.4316e+05,3.7778e+05,4.1404e+05,4.5193e+05,4.9146e+05,5.3261e+05,5.754e+05,6.1981e+05,6.6584e+05,7.135e+05,7.6278e+05,8.1368e+05,8.6619e+05,9.2032e+05,9.7607e+05,1.0334e+06,1.0924e+06,1.153e+06,1.2152e+06,1.279e+06,1.3444e+06,1.4114e+06,1.48e+06,1.5502e+06,1.6221e+06,1.6955e+06,1.7705e+06,1.8471e+06,1.9254e+06,2.0052e+06,2.0866e+06
      | 0,1024.5,4013.8,8921.9,15725,24406,34953,47356,61605,77694,95616,1.1537e+05,1.3694e+05,1.6032e+05,1.8553e+05,2.1254e+05,2.4135e+05,2.7197e+05,3.0438e+05,3.3859e+05,3.7459e+05,4.1238e+05,4.5196e+05,4.9333e+05,5.3647e+05,5.814e+05,6.281e+05,6.7658e+05,7.2683e+05,7.7885e+05,8.3264e+05,8.8821e+05,9.4553e+05,1.0046e+06,1.0655e+06,1.1281e+06,1.1925e+06,1.2586e+06,1.3265e+06,1.3961e+06,1.4675e+06,1.5407e+06,1.6156e+06,1.6922e+06,1.7706e+06,1.8508e+06,1.9327e+06,2.0163e+06,2.1017e+06,2.1889e+06,2.2777e+06
      | 0,1114.7,4367.1,9707.2,17109,26554,38030,51524,67028,84533,1.0403e+05,1.2552e+05,1.4899e+05,1.7444e+05,2.0185e+05,2.3124e+05,2.6259e+05,2.959e+05,3.3117e+05,3.6839e+05,4.0756e+05,4.4868e+05,4.9174e+05,5.3675e+05,5.8369e+05,6.3257e+05,6.8338e+05,7.3613e+05,7.908e+05,8.474e+05,9.0593e+05,9.6638e+05,1.0288e+06,1.093e+06,1.1593e+06,1.2274e+06,1.2974e+06,1.3694e+06,1.4432e+06,1.519e+06,1.5967e+06,1.6763e+06,1.7578e+06,1.8412e+06,1.9265e+06,2.0137e+06,2.1028e+06,2.1938e+06,2.2867e+06,2.3815e+06,2.4782e+06]
  Terminator{,1..6} (7 alike) : Terminator
  Wheel : Outport  VectorParamsAs1DForOutWhenUnconnected=off
  wires:
  Fiala Tire/1 -> Wheel/1
  Camber/1 -> Fiala Tire/5
  r/1 -> Fiala Tire/6
  Vy/1 -> Fiala Tire/4
  AxlTrq/1 -> Fiala Tire/2
  BrkPrs/1 -> Fiala Tire/1
  Vx/1 -> Fiala Tire/3
  TirePrs/1 -> Fiala Tire/7
  Ground/1 -> Fiala Tire/8
  Fz/1 -> Fiala Tire/9
  Friction/1 -> Fiala Tire/10
  Fiala Tire/2 -> Terminator/1
  Fiala Tire/3 -> Terminator1/1
  Fiala Tire/5 -> Terminator3/1
  Fiala Tire/4 -> Terminator2/1
  Fiala Tire/8 -> Terminator6/1
  Fiala Tire/7 -> Terminator5/1
  Fiala Tire/6 -> Terminator4/1

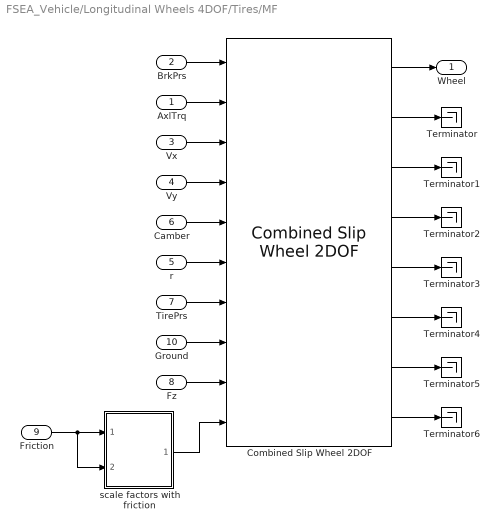
== system FSEA_Vehicle/Longitudinal Wheels 4DOF/Tires/MF ==
  AxlTrq : Inport
  BrkPrs : Inport  Port=2
  Vx : Inport  Port=3
  Vy : Inport  Port=4
  r : Inport  Port=5
  Camber : Inport  Port=6
  TirePrs : Inport  Port=7
  Fz : Inport  Port=8
  Friction : Inport  Port=9
  Ground : Inport  Port=10
  Combined Slip Wheel 2DOF : vehdynlibtire/Combined Slip Wheel 2DOF  tireType=Mid-size passenger car 235/45R18  tireParamSet=vdynPassCar.mat  vertType=None  plySteer=off  turnslip=off  BrakeType=Disc  mu_static=.3  mu_kinetic=.2  drum_abore=0.0508  drum_a=0.123  drum_c=0.212  drum_r=0.15  drum_theta1=0  drum_theta2=126  disk_abore=.05  Rm=.177  num_pads=2  brake_p_bpt=[1 11.4736842105263 21.9473684210526 32.4210526315789 42.8947368421053 53.3684210526316 63.8421052631579 74.3157894736842 84.7894736842105 95.2631578947368 105.736842105263 116.210526315789 126.684210526316 137.157894736842 147.631578947368 158.105263157895 168.578947368421 179.052631578947 189.526315789474 200]  brake_n_bpt=[0 52.6315789473684 105.263157894737 157.894736842105 210.526315789474 263.157894736842 315.789473684211 368.421052631579 421.052631578947 473.684210526316 526.315789473684 578.947368421053 631.578947368421 684.210526315789 736.842105263158 789.473684210526 842.105263157895 894.736842105263 947.368421052632 1000]  f_brake_t=[43.4900602404453 42.5056030554862 41.5350898940194 40.5780454442085 39.6340111501808 38.7025443887544 37.7832176914519 36.8756180088306 35.9793460143796 35.0940154454303 34.2192524787115 33.3546951383474 32.4999927342521 31.6548053290159 30.8188032315107 29.991666515561 29.1730845621415 28.362755623661 27.5603864089927 26.765691687993;498.991217495636 487.695866636631 476.560505099801 465.579679307235 454.748127933653 444.060772460445 433.51270824929 423.099196101319 412.81565427025 402.657650900201 392.620896861006 382.701238955775 372.894653477208 363.197240090814 353.605216024701 344.114910546964 334.722759712992 325.425301366216 316.219170376863 307.10109410434;954.492374750826 932.886130217776 911.585920305583 890.581313170261 869.862244717126 849.419000532136 829.242198807128 809.322774193808 789.651962526121 770.221286354971 751.0225412433 732.047782773203 713.289314220164 694.739674852612 676.391628817892 658.238154578366 640.272434863842 622.48784710877 604.877954344734 587.436496520688;1409.99353200602 1378.07639379892 1346.61133551136 1315.58294703329 1284.9763615006 1254.77722860383 1224.97168936497 1195.5463522863 1166.48827078199 1137.78492180974 1109.42418562559 1081.39432659063 1053.68397496312 1026.28210961441 999.178041611083 972.361398609768 945.822110014692 919.550392851325 893.536738312604 867.771898937035;1865.49468926121 1823.26665738007 1781.63675071715 1740.58458089631 1700.09047828407 1660.13545667552 1620.7011799228 1581.76993037878 1543.32457903786 1505.34855726451 1467.82583000789 1430.74087040806 1394.07863570608 1357.82454437621 1321.96445440427 1286.48464264117 1251.37178516554 1216.61293859388 1182.19552228048 1148.10730135338;2320.9958465164 2268.45692096121 2216.66216592293 2165.58621475934 2115.20459506754 2065.49368474721 2016.43067048064 1967.99350847127 1920.16088729373 1872.91219271928 1826.22747439018 1780.08741422549 1734.47329644903 1689.36697913801 1644.75086719747 1600.60788667257 1556.92146031639 1513.67548433643 1470.85430624835 1428.44270376973;2776.49700377159 2713.64718454235 2651.68758112871 2590.58784862237 2530.31871185102 2470.8519128189 2412.16016103848 2354.21708656376 2296.9971955496 2240.47582817405 2184.62911877248 2129.43395804292 2074.86795719199 2020.9094138998 1967.53727999066 1914.73113070398 1862.47113546724 1810.73803007899 1759.51309021622 1708.77810618608;3231.99816102678 3158.8374481235 3086.71299633449 3015.58948248539 2945.43282863449 2876.21014089059 2807.88965159632 2740.44066465625 2673.83350380547 2608.03946362882 2543.03076315477 2478.78050186034 2415.26261793494 2352.4518486616 2290.32369278385 2228.85437473538 2168.02081061809 2107.80057582154 2048.17187418409 1989.11350860242;3687.49931828197 3604.02771170464 3521.73841154027 3440.59111634842 3360.54694541796 3281.56836896228 3203.61914215416 3126.66424274874 3050.66981206134 2975.60309908359 2901.43240753707 2828.12704567777 2755.6572786779 2683.9942834234 2613.11010557704 2542.97761876678 2473.57048576894 2404.8631215641 2336.83065815196 2269.44891101877;4143.00047553716 4049.21797528579 3956.76382674606 3865.59275021144 3775.66106220143 3686.92659703397 3599.34863271199 3512.88782084123 3427.50612031721 3343.16673453836 3259.83405191936 3177.4735894952 3096.05193942085 3015.5367181852 2935.89651837023 2857.10086279818 2779.12016091979 2701.92566730665 2625.48944211983 2549.78431343512;4598.50163279235 4494.40823886693 4391.78924195184 4290.59438407447 4190.77517898491 4092.28482510566 3995.07812326983 3899.11139893372 3804.34242857308 3710.73036999313 3618.23569630166 3526.82013331263 3436.44660016381 3347.079152947 3258.68293116342 3171.22410682959 3084.66983607064 2998.98821304921 2914.1482260877 2830.11971585147;5054.00279004754 4939.59850244808 4826.81465715762 4715.59601793749 4605.88929576838 4497.64305317735 4390.80761382767 4285.3349770262 4181.17873682896 4078.2940054479 3976.63734068395 3876.16667713006 3776.84126090677 3678.62158770879 3581.46934395661 3485.34735086099 ...(+2764 chars)]  NOMPRES=262000  PRESMAX=1000000  PRESMIN=10000  FNOMIN=4300  FZMAX=8600  FZMIN=100  VXLOW=1  KPUMAX=1.5  KPUMIN=-1.5  ALPMAX=1.5  ALPMIN=-1.5  CAMMAX=0.17453  CAMMIN=-0.17453  LONGVL=16.7  FxRelFreqLwrLim=40*pi  FyRelFreqLwrLim=0  MyRelFreqLwrLim=40*pi  omegao=0  UNLOADED_RADIUS=0.33454  WIDTH=0.235  RIM_RADIUS=0.2286  ASPECT_RATIO=0.45  MASS=11.2  IYY=1.084  br=1e-3  GRAVITY=-9.81  zo=.015+VEH.InitialVertPosition  zdoto=0  BREFF=8.25094594147963  DREFF=0.260468730454265  FREFF=0.0735298544471851  Q_RE0=1.00866439868088  Q_V1=0.000760413786224011  Q_V2=0.0463384792019201  Q_FZ1=0  Q_FZ2=15.6870832810226  Q_FZ3=0  Q_FCX=0.138643970247602  Q_FCY=0.10843499565426  Q_FCY2=-0.465763352339538  PFZ1=0.69958166705601  VERTICAL_STIFFNESS=207885.061134007  VERTICAL_DAMPING=500  BOTTOM_OFFST=0.00990653336182505  BOTTOM_STIFF=1999075.87051971  Q_CAM1=86.7791723017291  Q_CAM2=259.705254231766  Q_CAM3=0.510281667378416  Q_FYS1=-20769.4728880343  Q_FYS2=-59060.183485617  Q_FYS3=89271.8260126986  LONGITUDINAL_STIFFNESS=388714.175879854  LATERAL_STIFFNESS=157087.404633332  PCFX1=0.18539229191199  PCFX2=0  PCFX3=0  PCFY1=0.163183345037677  PCFY2=0  PCFY3=0.249094918231954  Q_RA1=0.675942571700787  Q_RA2=0.73800463546164  Q_RB1=1.04487486456705  Q_RB2=-1.191763806629  PCX1=1.58523057950359  PDX1=1.0239116238178  PDX2=-0.0842405110022724  PDX3=0  PEX1=0.110312777158455  PEX2=0.313468516038146  PEX3=0  PEX4=0.0016060905760045  PKX1=21.3872544684023  PKX2=14.0006541873175  PKX3=-0.405326109653452  PHX1=0.000212599305364818  PHX2=0.00115950515263055  PVX1=1.59236164471432e-05  PVX2=0.000104321112127671  PPX1=-0.349461321276586  PPX2=0.387840040616429  PPX3=-0.0969947336569324  PPX4=0.0632271859795801  RBX1=12.7633329850276  RBX2=9.5787123658471  RBX3=0  RCX1=1.02796280922059  REX1=-0.45202516851367  REX2=-0.47304886171176  RHX1=0.000233272373115809  QSX1=-0.00788307788961443  QSX2=0.954629515459396  QSX3=0.0155855777667025  QSX4=0.125904607142414  QSX5=1.01110069703963  QSX6=20.1938577118433  QSX7=0.310818120717083  QSX8=-0.0430823751139655  QSX9=0.636494404888216  QSX10=0.142438060591663  QSX11=0.346766530036373  QSX12=0  QSX13=0  QSX14=0  PPMX1=0  PCY1=1.34299950037631  PDY1=0.878267729082195  PDY2=-0.0644597923147385  PDY3=0  PEY1=-0.809776534470972  PEY2=-0.600180598867198  PEY3=0.0991732552633487  PEY4=-6.5577974035573  PEY5=0  PKY1=-15.5714726518315  PKY2=1.73126522291751  PKY3=0.365349873517229  PKY4=1.98176755955416  PKY5=0  PKY6=-0.884005199550313  PKY7=-0.237259727611847  PHY1=-0.00183370557235628  PHY2=0.00346401302716671  PVY1=-0.00675427560163264  PVY2=0.036379218103843  PVY3=-0.163543984089166  PVY4=-0.491003349625726  PPY1=-0.62059646553185  PPY2=-0.0647824842338686  PPY3=-0.164648843290686  PPY4=0.283193909060098  PPY5=0  RBY1=10.7588809173639  RBY2=7.70420065295029  RBY3=3.40283755070691e-06  RBY4=0  RCY1=1.06691874059059  REY1=0.308244924574305  REY2=7.48775032604508e-06  RHY1=0.0118479204960415  RHY2=7.63650177161071e-06  RVY1=0.0560024425050078  RVY2=7.48487127056197e-06  RVY3=0  RVY4=98.4047026517149  RVY5=2.02759273900054  RVY6=15.7623064923347  QSY1=0.00699077564863536  QSY2=0  QSY3=0.00153535478298811  QSY4=8.55710322455322e-05  QSY5=0  QSY6=0  QSY7=0.89443879773793  QSY8=-0.403227641260894  QBZ1=11.666656027484  QBZ2=-1.30355438574485  QBZ3=0  QBZ4=0.177918305399071  QBZ5=-0.162481135068033  QBZ6=0  QBZ9=30.1445534682089  QBZ10=0  QCZ1=1.29026978207574  QDZ1=0.0886972644991399  QDZ2=-0.0058634820161856  QDZ3=0.3805597481383  QDZ4=0  QDZ6=0.00160914918118959  QDZ7=-0.00211036330862154  QDZ8=-0.13921904912557  QDZ9=0.00816585550028243  QDZ10=0  QDZ11=0  QEZ1=-2.19802254534746  QEZ2=1.01850535789165  QEZ3=0  QEZ4=0.278379679112054  QEZ5=-0.548414722765386  QHZ1=0.00148361198869669  QHZ2=0.00202017567585904  QHZ3=0.240316641332066  QHZ4=-0.210114035738085  PPZ1=-0.443927982388615  PPZ2=0  SSZ1=0.00914999585397887  SSZ2=0.0389830656052735  SSZ3=0  SSZ4=0  PDXP1=0.396718274678791  PDXP2=0  PDXP3=0  PKYP1=1.00587060633573  PDYP1=0.40483048923438  PDYP2=0  PDYP3=0  PDYP4=0  PHYP1=0.992731942067188  PHYP2=0.150352945499914  PHYP3=0  PHYP4=-3.98988682633674  PECP1=0.502379254513503  PECP2=0  QDTP1=10.0178654287947  QCRP1=0.200627747200702  QCRP2=0.0995735881599772  QBRP1=0.0997107127960717  QDRP1=1.01432910167423  QDRP2=0  aMode=2
  Terminator{,1..6} (7 alike) : Terminator
  scale factors with friction : Subsystem  mask{numWheels=4}
      mask prompts: numWheels "Number of wheels"
  Wheel : Outport  VectorParamsAs1DForOutWhenUnconnected=off
  wires:
  Combined Slip Wheel 2DOF/6 -> Terminator4/1
  Combined Slip Wheel 2DOF/7 -> Terminator5/1
  Combined Slip Wheel 2DOF/8 -> Terminator6/1
  Combined Slip Wheel 2DOF/4 -> Terminator2/1
  Combined Slip Wheel 2DOF/5 -> Terminator3/1
  Combined Slip Wheel 2DOF/3 -> Terminator1/1
  Combined Slip Wheel 2DOF/2 -> Terminator/1
  Fz/1 -> Combined Slip Wheel 2DOF/9
  Ground/1 -> Combined Slip Wheel 2DOF/8
  TirePrs/1 -> Combined Slip Wheel 2DOF/7
  Vx/1 -> Combined Slip Wheel 2DOF/3
  BrkPrs/1 -> Combined Slip Wheel 2DOF/1
  AxlTrq/1 -> Combined Slip Wheel 2DOF/2
  Vy/1 -> Combined Slip Wheel 2DOF/4
  r/1 -> Combined Slip Wheel 2DOF/6
  Camber/1 -> Combined Slip Wheel 2DOF/5
  Combined Slip Wheel 2DOF/1 -> Wheel/1
  Friction/1 -> scale factors with friction/2(lamda_mu_y), scale factors with friction/1(lamda_mu_x)
  scale factors with friction/1(lambdas) -> Combined Slip Wheel 2DOF/10
